simulink subsystem "PreliminaryServo"  (R2025b)
settings: Solver=VariableStepAuto  StartTime=0.0  StopTime=10.0  RelTol=1e-3
libraries: robotmaniplib x1
settings Model: Creator=Compu  LastModifiedBy=Compu

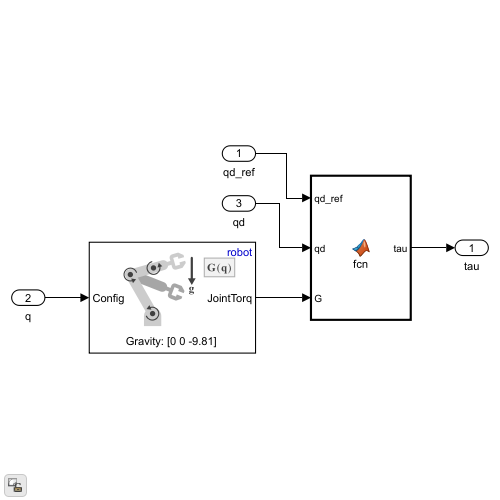
[thumbnail: Simulink's stored preview of the top-level diagram]
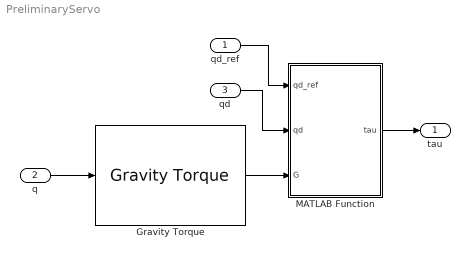
== system PreliminaryServo ==
  qd_ref : Inport
  q : Inport  Port=2
  qd : Inport  Port=3
  Gravity Torque : robotmaniplib/Gravity Torque  RigidBodyTree=robot  SimulateUsing=Interpreted execution
  MATLAB Function : MATLAB Function  TreatAsAtomicUnit=on
  tau : Outport
  wires:
  MATLAB Function/1(tau) -> tau/1
  q/1 -> Gravity Torque/1
  qd_ref/1 -> MATLAB Function/1(qd_ref)
  Gravity Torque/1 -> MATLAB Function/3(G)
  qd/1 -> MATLAB Function/2(qd)

== matlab function PreliminaryServo/MATLAB Function ==
  data: qd_ref input; qd input; G input; tau output size=[6 1]; Kv_servo parameter
function tau = fcn(qd_ref,qd,G,Kv_servo)
% Preliminary joint velocity servo.

qd_ref = reshape(qd_ref,6,1);
qd     = reshape(qd,6,1);
G      = reshape(G,6,1);

% Velocity tracking error.
e = qd_ref - qd;

% Commanded joint torque [Nm].
tau = Kv_servo(:).*e + G;

end
